simulink model "AFC_FFNN_trainbfg_60_60_60_Nor_July_15_Rep"  (R2021a)
settings: Solver=ode15s  StartTime=0.0  StopTime=T  MaxStep=.01  RelTol=1e-3
undefined symbols (not defined in the file): AF_sensor_tol, fault_time, fuel_inj_tol, kappa_tol, MAF_sensor_tol, pump_tol, tau_ww_tol, Ts, x_gain, x_offset, y_gain, y_offset
libraries: neural x185, dspsrcs4 x3
(part 2 of 8)

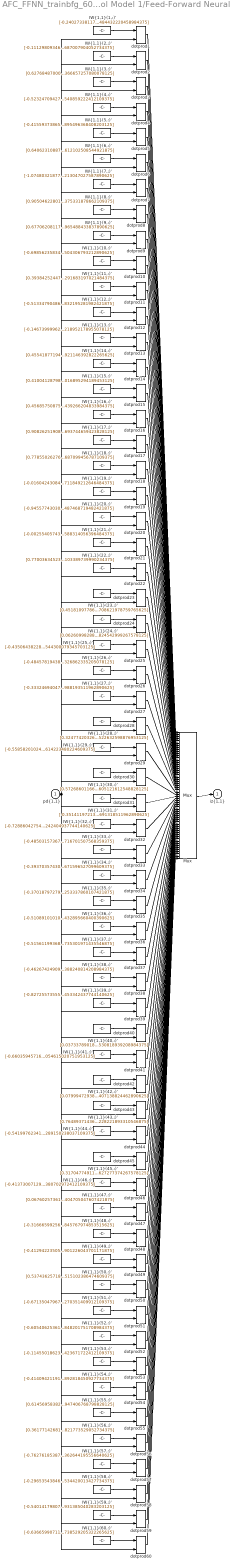
== system AFC_FFNN_trainbfg_60_60_60_Nor_July_15_Rep/Air Fuel Control Model 1/Feed-Forward Neural Network/Layer 1/IW{1,1} ==
  "pd{1,1}" : Inport  PortDimensions=4
      mask Display: e = 0.06;c1 = [120 230 180]/255;c2 = ([120 230 180]+0)/(256+128);c3 = ([120 230 180]+128)/(256+128);patch([0 1 1 0],[0 0 1 1],c1);patch([0 1 1 1-e 1-e 0+e],[0 0 1 1-e 0+e 0+e],c2);patch([0 0 1 1-e 0+e 0+e],[0 1 1 1-e 1-e 0+e],c3);plot([0 1 1 0 0],[0 0 1 1 0]);
  "IW{1,1}(1,:)'" : Constant  Value=[-0.2402733811760711102323284649173729121685028076171875;0.0584441094356973334100757710984908044338226318359375;-0.6963364088024845965918530055205337703227996826171875;-0.288781535204351680334866614430211484432220458984375]
      mask Display: e = 0.06;c1 = [120 150 230]/255;c2 = ([120 150 230]+0)/383;c3 = ([120 150 230]+128)/383;patch([0 1 1 0],[0 0 1 1],c1);patch([0 1 1 1-e 1-e 0+e],[0 0 1 1-e 0+e 0+e],c2);patch([0 0 1 1-e 0+e 0+e],[0 1 1 1-e 1-e 0+e],c3);plot([0 1 1 0 0],[0 0 1 1 0]);disp('Weights');
  "IW{1,1}(10,:)'" : Constant  Value=[-0.698562358345947043147816657437942922115325927734375;0.69054064531703496232495353979174979031085968017578125;-0.18905586459529022391734542907215654850006103515625;-0.91927275641961225804976720610284246504306793212890625]
      mask Display: e = 0.06;c1 = [120 150 230]/255;c2 = ([120 150 230]+0)/383;c3 = ([120 150 230]+128)/383;patch([0 1 1 0],[0 0 1 1],c1);patch([0 1 1 1-e 1-e 0+e],[0 0 1 1-e 0+e 0+e],c2);patch([0 0 1 1-e 0+e 0+e],[0 1 1 1-e 1-e 0+e],c3);plot([0 1 1 0 0],[0 0 1 1 0]);disp('Weights');
  "IW{1,1}(11,:)'" : Constant  Value=[0.39384252447863554724705181797617115080356597900390625;-0.0292738838791086024293530698514587129466235637664794921875;0.58197351258983232025201459691743366420269012451171875;0.8598468943954189480649574761628173291683197021484375]
      mask Display: e = 0.06;c1 = [120 150 230]/255;c2 = ([120 150 230]+0)/383;c3 = ([120 150 230]+128)/383;patch([0 1 1 0],[0 0 1 1],c1);patch([0 1 1 1-e 1-e 0+e],[0 0 1 1-e 0+e 0+e],c2);patch([0 0 1 1-e 0+e 0+e],[0 1 1 1-e 1-e 0+e],c3);plot([0 1 1 0 0],[0 0 1 1 0]);disp('Weights');
  "IW{1,1}(12,:)'" : Constant  Value=[-0.513347904862785586743711974122561514377593994140625;-0.869373002560909657887577850488014519214630126953125;0.72775650268875191617468090043985284864902496337890625;0.47288176623451583235890893774922005832195281982421875]
      mask Display: e = 0.06;c1 = [120 150 230]/255;c2 = ([120 150 230]+0)/383;c3 = ([120 150 230]+128)/383;patch([0 1 1 0],[0 0 1 1],c1);patch([0 1 1 1-e 1-e 0+e],[0 0 1 1-e 0+e 0+e],c2);patch([0 0 1 1-e 0+e 0+e],[0 1 1 1-e 1-e 0+e],c3);plot([0 1 1 0 0],[0 0 1 1 0]);disp('Weights');
  "IW{1,1}(13,:)'" : Constant  Value=[-0.1467399996214004131989128154600621201097965240478515625;-0.249808478302043723839886979476432316005229949951171875;0.507943904783524136092864864622242748737335205078125;0.71026397639314087228967764531262218952178955078125]
      mask Display: e = 0.06;c1 = [120 150 230]/255;c2 = ([120 150 230]+0)/383;c3 = ([120 150 230]+128)/383;patch([0 1 1 0],[0 0 1 1],c1);patch([0 1 1 1-e 1-e 0+e],[0 0 1 1-e 0+e 0+e],c2);patch([0 0 1 1-e 0+e 0+e],[0 1 1 1-e 1-e 0+e],c3);plot([0 1 1 0 0],[0 0 1 1 0]);disp('Weights');
  "IW{1,1}(14,:)'" : Constant  Value=[0.4554187719467928108230125872069038450717926025390625;0.411659817080715140225066761558991856873035430908203125;0.2102615703971319194298672528020688332617282867431640625;-0.322493540823335200773414044306264258921146392822265625]
      mask Display: e = 0.06;c1 = [120 150 230]/255;c2 = ([120 150 230]+0)/383;c3 = ([120 150 230]+128)/383;patch([0 1 1 0],[0 0 1 1],c1);patch([0 1 1 1-e 1-e 0+e],[0 0 1 1-e 0+e 0+e],c2);patch([0 0 1 1-e 0+e 0+e],[0 1 1 1-e 1-e 0+e],c3);plot([0 1 1 0 0],[0 0 1 1 0]);disp('Weights');
  "IW{1,1}(15,:)'" : Constant  Value=[0.410041287982604085726734410854987800121307373046875;0.531329072729679108277878185617737472057342529296875;0.441581495936325563178570519085042178630828857421875;0.7428199021330688101016903601703234016895294189453125]
      mask Display: e = 0.06;c1 = [120 150 230]/255;c2 = ([120 150 230]+0)/383;c3 = ([120 150 230]+128)/383;patch([0 1 1 0],[0 0 1 1],c1);patch([0 1 1 1-e 1-e 0+e],[0 0 1 1-e 0+e 0+e],c2);patch([0 0 1 1-e 0+e 0+e],[0 1 1 1-e 1-e 0+e],c3);plot([0 1 1 0 0],[0 0 1 1 0]);disp('Weights');
  "IW{1,1}(16,:)'" : Constant  Value=[0.45685750875504094192791626483085565268993377685546875;-0.465586840801124945965483448162558488547801971435546875;-0.9097857307732315490511609823442995548248291015625;0.056854430973618828859539320319527178071439266204833984375]
      mask Display: e = 0.06;c1 = [120 150 230]/255;c2 = ([120 150 230]+0)/383;c3 = ([120 150 230]+128)/383;patch([0 1 1 0],[0 0 1 1],c1);patch([0 1 1 1-e 1-e 0+e],[0 0 1 1-e 0+e 0+e],c2);patch([0 0 1 1-e 0+e 0+e],[0 1 1 1-e 1-e 0+e],c3);plot([0 1 1 0 0],[0 0 1 1 0]);disp('Weights');
  "IW{1,1}(17,:)'" : Constant  Value=[0.90826251908224531206315077724866569042205810546875;-0.168991405620153134492511526332236826419830322265625;-0.3326678975694663531470496309339068830013275146484375;-0.2185158166571838922465076393564231693744659423828125]
      mask Display: e = 0.06;c1 = [120 150 230]/255;c2 = ([120 150 230]+0)/383;c3 = ([120 150 230]+128)/383;patch([0 1 1 0],[0 0 1 1],c1);patch([0 1 1 1-e 1-e 0+e],[0 0 1 1-e 0+e 0+e],c2);patch([0 0 1 1-e 0+e 0+e],[0 1 1 1-e 1-e 0+e],c3);plot([0 1 1 0 0],[0 0 1 1 0]);disp('Weights');
  "IW{1,1}(18,:)'" : Constant  Value=[0.77855026276990724198867610539309680461883544921875;0.5494533878008895921851717503159306943416595458984375;-0.19968633757158349428806332070962525904178619384765625;0.057413702447717838983631821747621870599687099456787109375]
      mask Display: e = 0.06;c1 = [120 150 230]/255;c2 = ([120 150 230]+0)/383;c3 = ([120 150 230]+128)/383;patch([0 1 1 0],[0 0 1 1],c1);patch([0 1 1 1-e 1-e 0+e],[0 0 1 1-e 0+e 0+e],c2);patch([0 0 1 1-e 0+e 0+e],[0 1 1 1-e 1-e 0+e],c3);plot([0 1 1 0 0],[0 0 1 1 0]);disp('Weights');
  "IW{1,1}(19,:)'" : Constant  Value=[-0.01604243084496127791371833382072509266436100006103515625;0.7508500028717011165468875333317555487155914306640625;0.702339376844223206575179574429057538509368896484375;-0.96384498936832496696069938479922711849212646484375]
      mask Display: e = 0.06;c1 = [120 150 230]/255;c2 = ([120 150 230]+0)/383;c3 = ([120 150 230]+128)/383;patch([0 1 1 0],[0 0 1 1],c1);patch([0 1 1 1-e 1-e 0+e],[0 0 1 1-e 0+e 0+e],c2);patch([0 0 1 1-e 0+e 0+e],[0 1 1 1-e 1-e 0+e],c3);plot([0 1 1 0 0],[0 0 1 1 0]);disp('Weights');
  "IW{1,1}(2,:)'" : Constant  Value=[-0.11129809346802523040143029220416792668402194976806640625;1.19471297517650665298560852534137666225433349609375;0.8221228609018293997934279104811139404773712158203125;0.261811524571846143683018226511194370687007904052734375]
      mask Display: e = 0.06;c1 = [120 150 230]/255;c2 = ([120 150 230]+0)/383;c3 = ([120 150 230]+128)/383;patch([0 1 1 0],[0 0 1 1],c1);patch([0 1 1 1-e 1-e 0+e],[0 0 1 1-e 0+e 0+e],c2);patch([0 0 1 1-e 0+e 0+e],[0 1 1 1-e 1-e 0+e],c3);plot([0 1 1 0 0],[0 0 1 1 0]);disp('Weights');
  "IW{1,1}(20,:)'" : Constant  Value=[-0.945577430309771482797032149392180144786834716796875;-0.6815723884271618349117716206819750368595123291015625;0.3251297032677182841098328935913741588592529296875;-0.27675916067568884226801628756220452487468719482421875]
      mask Display: e = 0.06;c1 = [120 150 230]/255;c2 = ([120 150 230]+0)/383;c3 = ([120 150 230]+128)/383;patch([0 1 1 0],[0 0 1 1],c1);patch([0 1 1 1-e 1-e 0+e],[0 0 1 1-e 0+e 0+e],c2);patch([0 0 1 1-e 0+e 0+e],[0 1 1 1-e 1-e 0+e],c3);plot([0 1 1 0 0],[0 0 1 1 0]);disp('Weights');
  "IW{1,1}(21,:)'" : Constant  Value=[-0.0025540574341372016507756281811225562705658376216888427734375;-0.9119172902964922666768643466639332473278045654296875;-0.10602108765426902781126017316637444309890270233154296875;0.9466934496951624478100484338938258588314056396484375]
      mask Display: e = 0.06;c1 = [120 150 230]/255;c2 = ([120 150 230]+0)/383;c3 = ([120 150 230]+128)/383;patch([0 1 1 0],[0 0 1 1],c1);patch([0 1 1 1-e 1-e 0+e],[0 0 1 1-e 0+e 0+e],c2);patch([0 0 1 1-e 0+e 0+e],[0 1 1 1-e 1-e 0+e],c3);plot([0 1 1 0 0],[0 0 1 1 0]);disp('Weights');
  "IW{1,1}(22,:)'" : Constant  Value=[0.77003634523305664050241148288478143513202667236328125;0.5101538838642649675847451362642459571361541748046875;1.2853720282784777406703824453870765864849090576171875;-0.3114234464103569077764177563949488103389739990234375]
      mask Display: e = 0.06;c1 = [120 150 230]/255;c2 = ([120 150 230]+0)/383;c3 = ([120 150 230]+128)/383;patch([0 1 1 0],[0 0 1 1],c1);patch([0 1 1 1-e 1-e 0+e],[0 0 1 1-e 0+e 0+e],c2);patch([0 0 1 1-e 0+e 0+e],[0 1 1 1-e 1-e 0+e],c3);plot([0 1 1 0 0],[0 0 1 1 0]);disp('Weights');
  "IW{1,1}(23,:)'" : Constant  Value=[0.451810977860063023303638374272850342094898223876953125;0.97595879998877788086275586465490050613880157470703125;-1.0004027544089548751315987829002551734447479248046875;0.425110540617065046919975657147006131708621978759765625]
      mask Display: e = 0.06;c1 = [120 150 230]/255;c2 = ([120 150 230]+0)/383;c3 = ([120 150 230]+128)/383;patch([0 1 1 0],[0 0 1 1],c1);patch([0 1 1 1-e 1-e 0+e],[0 0 1 1-e 0+e 0+e],c2);patch([0 0 1 1-e 0+e 0+e],[0 1 1 1-e 1-e 0+e],c3);plot([0 1 1 0 0],[0 0 1 1 0]);disp('Weights');
  "IW{1,1}(24,:)'" : Constant  Value=[0.06260998288320009097507323758691200055181980133056640625;0.70118255617086788777925221438636071979999542236328125;-0.41558101347191478414089260695618577301502227783203125;-0.8023807819065560398286152121727354824542999267578125]
      mask Display: e = 0.06;c1 = [120 150 230]/255;c2 = ([120 150 230]+0)/383;c3 = ([120 150 230]+128)/383;patch([0 1 1 0],[0 0 1 1],c1);patch([0 1 1 1-e 1-e 0+e],[0 0 1 1-e 0+e 0+e],c2);patch([0 0 1 1-e 0+e 0+e],[0 1 1 1-e 1-e 0+e],c3);plot([0 1 1 0 0],[0 0 1 1 0]);disp('Weights');
  "IW{1,1}(25,:)'" : Constant  Value=[-0.43506438228140986712588755835895426571369171142578125;-1.10068797433876230940086315968073904514312744140625;0.58386265727177566464689562053536064922809600830078125;0.3360856882674394530141626091790385544300079345703125]
      mask Display: e = 0.06;c1 = [120 150 230]/255;c2 = ([120 150 230]+0)/383;c3 = ([120 150 230]+128)/383;patch([0 1 1 0],[0 0 1 1],c1);patch([0 1 1 1-e 1-e 0+e],[0 0 1 1-e 0+e 0+e],c2);patch([0 0 1 1-e 0+e 0+e],[0 1 1 1-e 1-e 0+e],c3);plot([0 1 1 0 0],[0 0 1 1 0]);disp('Weights');
  "IW{1,1}(26,:)'" : Constant  Value=[-0.484578194384843730091461111442185938358306884765625;0.08274506282760592246194875087894615717232227325439453125;0.266533819315904363378422203822992742061614990234375;-0.444300663044444654747877621048246510326862335205078125]
      mask Display: e = 0.06;c1 = [120 150 230]/255;c2 = ([120 150 230]+0)/383;c3 = ([120 150 230]+128)/383;patch([0 1 1 0],[0 0 1 1],c1);patch([0 1 1 1-e 1-e 0+e],[0 0 1 1-e 0+e 0+e],c2);patch([0 0 1 1-e 0+e 0+e],[0 1 1 1-e 1-e 0+e],c3);plot([0 1 1 0 0],[0 0 1 1 0]);disp('Weights');
  "IW{1,1}(27,:)'" : Constant  Value=[-0.333246940473589159381617719191126525402069091796875;0.620357973300408982453291173442266881465911865234375;-0.76705337279785357207373408527928404510021209716796875;0.93596136081508130022399427616619504988193511962890625]
      mask Display: e = 0.06;c1 = [120 150 230]/255;c2 = ([120 150 230]+0)/383;c3 = ([120 150 230]+128)/383;patch([0 1 1 0],[0 0 1 1],c1);patch([0 1 1 1-e 1-e 0+e],[0 0 1 1-e 0+e 0+e],c2);patch([0 0 1 1-e 0+e 0+e],[0 1 1 1-e 1-e 0+e],c3);plot([0 1 1 0 0],[0 0 1 1 0]);disp('Weights');
  "IW{1,1}(28,:)'" : Constant  Value=[0.324774203262355898313984425840317271649837493896484375;-0.321182382515287800917036520331748761236667633056640625;0.086974910188199194838176708799437619745731353759765625;0.51123135063906322006488380793598480522632598876953125]
      mask Display: e = 0.06;c1 = [120 150 230]/255;c2 = ([120 150 230]+0)/383;c3 = ([120 150 230]+128)/383;patch([0 1 1 0],[0 0 1 1],c1);patch([0 1 1 1-e 1-e 0+e],[0 0 1 1-e 0+e 0+e],c2);patch([0 0 1 1-e 0+e 0+e],[0 1 1 1-e 1-e 0+e],c3);plot([0 1 1 0 0],[0 0 1 1 0]);disp('Weights');
  "IW{1,1}(29,:)'" : Constant  Value=[-0.55858201024710985027610377073870040476322174072265625;0.75433144332418422539632274492760188877582550048828125;1.237291002285560548301646122126840054988861083984375;0.051530715501696099101192061198162264190614223480224609375]
      mask Display: e = 0.06;c1 = [120 150 230]/255;c2 = ([120 150 230]+0)/383;c3 = ([120 150 230]+128)/383;patch([0 1 1 0],[0 0 1 1],c1);patch([0 1 1 1-e 1-e 0+e],[0 0 1 1-e 0+e 0+e],c2);patch([0 0 1 1-e 0+e 0+e],[0 1 1 1-e 1-e 0+e],c3);plot([0 1 1 0 0],[0 0 1 1 0]);disp('Weights');
  "IW{1,1}(3,:)'" : Constant  Value=[0.62768487000840966771875173435546457767486572265625;-0.23395389022367485409859000355936586856842041015625;-0.7323866072763622891983459339826367795467376708984375;-0.43736410145401283244837031816132366657257080078125]
      mask Display: e = 0.06;c1 = [120 150 230]/255;c2 = ([120 150 230]+0)/383;c3 = ([120 150 230]+128)/383;patch([0 1 1 0],[0 0 1 1],c1);patch([0 1 1 1-e 1-e 0+e],[0 0 1 1-e 0+e 0+e],c2);patch([0 0 1 1-e 0+e 0+e],[0 1 1 1-e 1-e 0+e],c3);plot([0 1 1 0 0],[0 0 1 1 0]);disp('Weights');
  "IW{1,1}(30,:)'" : Constant  Value=[0.57268601166601029728298044574330560863018035888671875;0.5351151798944560056270347558893263339996337890625;0.6025777522967918908847195780253969132900238037109375;-0.4208352769974184059975641503115184605121612548828125]
      mask Display: e = 0.06;c1 = [120 150 230]/255;c2 = ([120 150 230]+0)/383;c3 = ([120 150 230]+128)/383;patch([0 1 1 0],[0 0 1 1],c1);patch([0 1 1 1-e 1-e 0+e],[0 0 1 1-e 0+e 0+e],c2);patch([0 0 1 1-e 0+e 0+e],[0 1 1 1-e 1-e 0+e],c3);plot([0 1 1 0 0],[0 0 1 1 0]);disp('Weights');
  "IW{1,1}(31,:)'" : Constant  Value=[-0.351411972139949624338584044380695559084415435791015625;-0.58862397289580592474322884299908764660358428955078125;0.405848519913738992048735099160694517195224761962890625;0.778774721855601370634758495725691318511962890625]
      mask Display: e = 0.06;c1 = [120 150 230]/255;c2 = ([120 150 230]+0)/383;c3 = ([120 150 230]+128)/383;patch([0 1 1 0],[0 0 1 1],c1);patch([0 1 1 1-e 1-e 0+e],[0 0 1 1-e 0+e 0+e],c2);patch([0 0 1 1-e 0+e 0+e],[0 1 1 1-e 1-e 0+e],c3);plot([0 1 1 0 0],[0 0 1 1 0]);disp('Weights');
  "IW{1,1}(32,:)'" : Constant  Value=[-0.7288604275436771917640044193831272423267364501953125;-0.996691557863663479821525470470078289508819580078125;0.433393450161783932994552515083341859281063079833984375;-0.99673661414379299827714930870570242404937744140625]
      mask Display: e = 0.06;c1 = [120 150 230]/255;c2 = ([120 150 230]+0)/383;c3 = ([120 150 230]+128)/383;patch([0 1 1 0],[0 0 1 1],c1);patch([0 1 1 1-e 1-e 0+e],[0 0 1 1-e 0+e 0+e],c2);patch([0 0 1 1-e 0+e 0+e],[0 1 1 1-e 1-e 0+e],c3);plot([0 1 1 0 0],[0 0 1 1 0]);disp('Weights');
  "IW{1,1}(33,:)'" : Constant  Value=[-0.485031573670599680525583607959561049938201904296875;0.611012222465525223213944627786986529827117919921875;-0.83546688891837372903381719879689626395702362060546875;-0.81775281563621859959312132559716701507568359375]
      mask Display: e = 0.06;c1 = [120 150 230]/255;c2 = ([120 150 230]+0)/383;c3 = ([120 150 230]+128)/383;patch([0 1 1 0],[0 0 1 1],c1);patch([0 1 1 1-e 1-e 0+e],[0 0 1 1-e 0+e 0+e],c2);patch([0 0 1 1-e 0+e 0+e],[0 1 1 1-e 1-e 0+e],c3);plot([0 1 1 0 0],[0 0 1 1 0]);disp('Weights');
  "IW{1,1}(34,:)'" : Constant  Value=[-0.3937035743010410815401201034546829760074615478515625;0.12437679182351264739470053655168158002197742462158203125;-0.1559704725434329919409037756850011646747589111328125;-0.377894968173168199765399322131997905671596527099609375]
      mask Display: e = 0.06;c1 = [120 150 230]/255;c2 = ([120 150 230]+0)/383;c3 = ([120 150 230]+128)/383;patch([0 1 1 0],[0 0 1 1],c1);patch([0 1 1 1-e 1-e 0+e],[0 0 1 1-e 0+e 0+e],c2);patch([0 0 1 1-e 0+e 0+e],[0 1 1 1-e 1-e 0+e],c3);plot([0 1 1 0 0],[0 0 1 1 0]);disp('Weights');
  "IW{1,1}(35,:)'" : Constant  Value=[-0.370187972793248276648370165275991894304752349853515625;-0.7998130855513536641154814788023941218852996826171875;0.359795410640817603376007127735647372901439666748046875;-0.7383023080329642606756124223466031253337860107421875]
      mask Display: e = 0.06;c1 = [120 150 230]/255;c2 = ([120 150 230]+0)/383;c3 = ([120 150 230]+128)/383;patch([0 1 1 0],[0 0 1 1],c1);patch([0 1 1 1-e 1-e 0+e],[0 0 1 1-e 0+e 0+e],c2);patch([0 0 1 1-e 0+e 0+e],[0 1 1 1-e 1-e 0+e],c3);plot([0 1 1 0 0],[0 0 1 1 0]);disp('Weights');
  "IW{1,1}(36,:)'" : Constant  Value=[-0.51089101010404203151438196073286235332489013671875;-0.56318994359729479537435281599755398929119110107421875;-0.377415197921292355776046179016702808439731597900390625;0.024662139600768552549769907500376575626432895660400390625]
      mask Display: e = 0.06;c1 = [120 150 230]/255;c2 = ([120 150 230]+0)/383;c3 = ([120 150 230]+128)/383;patch([0 1 1 0],[0 0 1 1],c1);patch([0 1 1 1-e 1-e 0+e],[0 0 1 1-e 0+e 0+e],c2);patch([0 0 1 1-e 0+e 0+e],[0 1 1 1-e 1-e 0+e],c3);plot([0 1 1 0 0],[0 0 1 1 0]);disp('Weights');
  "IW{1,1}(37,:)'" : Constant  Value=[-0.51561199368180066215927581652067601680755615234375;0.77000536182291334785787739747320301830768585205078125;0.29882660214653433694564910183544270694255828857421875;0.04938437783104136780121251604214194230735301971435546875]
      mask Display: e = 0.06;c1 = [120 150 230]/255;c2 = ([120 150 230]+0)/383;c3 = ([120 150 230]+128)/383;patch([0 1 1 0],[0 0 1 1],c1);patch([0 1 1 1-e 1-e 0+e],[0 0 1 1-e 0+e 0+e],c2);patch([0 0 1 1-e 0+e 0+e],[0 1 1 1-e 1-e 0+e],c3);plot([0 1 1 0 0],[0 0 1 1 0]);disp('Weights');
  "IW{1,1}(38,:)'" : Constant  Value=[-0.462674249097232370697696524075581692159175872802734375;-0.20404535875965346125582300373935140669345855712890625;-0.643589688538109161441980177187360823154449462890625;0.172530502878537050914786732391803525388240814208984375]
      mask Display: e = 0.06;c1 = [120 150 230]/255;c2 = ([120 150 230]+0)/383;c3 = ([120 150 230]+128)/383;patch([0 1 1 0],[0 0 1 1],c1);patch([0 1 1 1-e 1-e 0+e],[0 0 1 1-e 0+e 0+e],c2);patch([0 0 1 1-e 0+e 0+e],[0 1 1 1-e 1-e 0+e],c3);plot([0 1 1 0 0],[0 0 1 1 0]);disp('Weights');
  "IW{1,1}(39,:)'" : Constant  Value=[-0.827255735558199756241037903237156569957733154296875;0.31768520899595087403355364585877396166324615478515625;-0.26820571117561098350989823302370496094226837158203125;0.78370361390073883800511111985542811453342437744140625]
      mask Display: e = 0.06;c1 = [120 150 230]/255;c2 = ([120 150 230]+0)/383;c3 = ([120 150 230]+128)/383;patch([0 1 1 0],[0 0 1 1],c1);patch([0 1 1 1-e 1-e 0+e],[0 0 1 1-e 0+e 0+e],c2);patch([0 0 1 1-e 0+e 0+e],[0 1 1 1-e 1-e 0+e],c3);plot([0 1 1 0 0],[0 0 1 1 0]);disp('Weights');
  "IW{1,1}(4,:)'" : Constant  Value=[-0.5232470942791049850484341732226312160491943359375;-0.6811423805727827573974764163722284138202667236328125;-0.610543497321023753698909786180593073368072509765625;-0.224003810896950650288772521889768540859222412109375]
      mask Display: e = 0.06;c1 = [120 150 230]/255;c2 = ([120 150 230]+0)/383;c3 = ([120 150 230]+128)/383;patch([0 1 1 0],[0 0 1 1],c1);patch([0 1 1 1-e 1-e 0+e],[0 0 1 1-e 0+e 0+e],c2);patch([0 0 1 1-e 0+e 0+e],[0 1 1 1-e 1-e 0+e],c3);plot([0 1 1 0 0],[0 0 1 1 0]);disp('Weights');
  "IW{1,1}(40,:)'" : Constant  Value=[0.0373378901805889729104137586546130478382110595703125;0.8513626591803109544542849107529036700725555419921875;-0.9283781102192214529367220166022889316082000732421875;-0.250683731280675115016265408485196530818939208984375]
      mask Display: e = 0.06;c1 = [120 150 230]/255;c2 = ([120 150 230]+0)/383;c3 = ([120 150 230]+128)/383;patch([0 1 1 0],[0 0 1 1],c1);patch([0 1 1 1-e 1-e 0+e],[0 0 1 1-e 0+e 0+e],c2);patch([0 0 1 1-e 0+e 0+e],[0 1 1 1-e 1-e 0+e],c3);plot([0 1 1 0 0],[0 0 1 1 0]);disp('Weights');
  "IW{1,1}(41,:)'" : Constant  Value=[-0.660359457166579399967076824395917356014251708984375;-0.9795941991072105725635310591314919292926788330078125;-0.922451670193998207736285621649585664272308349609375;-0.87504814362874316913121219840832054615020751953125]
      mask Display: e = 0.06;c1 = [120 150 230]/255;c2 = ([120 150 230]+0)/383;c3 = ([120 150 230]+128)/383;patch([0 1 1 0],[0 0 1 1],c1);patch([0 1 1 1-e 1-e 0+e],[0 0 1 1-e 0+e 0+e],c2);patch([0 0 1 1-e 0+e 0+e],[0 1 1 1-e 1-e 0+e],c3);plot([0 1 1 0 0],[0 0 1 1 0]);disp('Weights');
  "IW{1,1}(42,:)'" : Constant  Value=[0.0799947293830058914210212606121785938739776611328125;-0.01554714821110536604464869014918804168701171875;0.9410230983615124333852008930989541113376617431640625;-0.4172880678448687152837237590574659407138824462890625]
      mask Display: e = 0.06;c1 = [120 150 230]/255;c2 = ([120 150 230]+0)/383;c3 = ([120 150 230]+128)/383;patch([0 1 1 0],[0 0 1 1],c1);patch([0 1 1 1-e 1-e 0+e],[0 0 1 1-e 0+e 0+e],c2);patch([0 0 1 1-e 0+e 0+e],[0 1 1 1-e 1-e 0+e],c3);plot([0 1 1 0 0],[0 0 1 1 0]);disp('Weights');
  "IW{1,1}(43,:)'" : Constant  Value=[0.7648937143639376046166944433934986591339111328125;-0.79666736296628493096960710317944176495075225830078125;0.2269171319430184630139279988725320436060428619384765625;0.312073469378814916108666466243448667228221893310546875]
      mask Display: e = 0.06;c1 = [120 150 230]/255;c2 = ([120 150 230]+0)/383;c3 = ([120 150 230]+128)/383;patch([0 1 1 0],[0 0 1 1],c1);patch([0 1 1 1-e 1-e 0+e],[0 0 1 1-e 0+e 0+e],c2);patch([0 0 1 1-e 0+e 0+e],[0 1 1 1-e 1-e 0+e],c3);plot([0 1 1 0 0],[0 0 1 1 0]);disp('Weights');
  "IW{1,1}(44,:)'" : Constant  Value=[-0.54199762341520685282603153609670698642730712890625;-0.6779396341603811659837219849578104913234710693359375;-0.0205716676017042576773974360548891127109527587890625;-0.2567857149437704489258749163127504289150238037109375]
      mask Display: e = 0.06;c1 = [120 150 230]/255;c2 = ([120 150 230]+0)/383;c3 = ([120 150 230]+128)/383;patch([0 1 1 0],[0 0 1 1],c1);patch([0 1 1 1-e 1-e 0+e],[0 0 1 1-e 0+e 0+e],c2);patch([0 0 1 1-e 0+e 0+e],[0 1 1 1-e 1-e 0+e],c3);plot([0 1 1 0 0],[0 0 1 1 0]);disp('Weights');
  "IW{1,1}(45,:)'" : Constant  Value=[0.317047749110300036701204362543649040162563323974609375;-0.49922870142301134510631754892528988420963287353515625;0.6173835365827649024339507377590052783489227294921875;-0.86470722989512360801001022991840727627277374267578125]
      mask Display: e = 0.06;c1 = [120 150 230]/255;c2 = ([120 150 230]+0)/383;c3 = ([120 150 230]+128)/383;patch([0 1 1 0],[0 0 1 1],c1);patch([0 1 1 1-e 1-e 0+e],[0 0 1 1-e 0+e 0+e],c2);patch([0 0 1 1-e 0+e 0+e],[0 1 1 1-e 1-e 0+e],c3);plot([0 1 1 0 0],[0 0 1 1 0]);disp('Weights');
  "IW{1,1}(46,:)'" : Constant  Value=[-0.41373007129052374875044506552512757480144500732421875;-0.4215260072473479002752583255642093718051910400390625;1.0491347537545305801387485189479775726795196533203125;-0.5364939166190045849447187720215879380702972412109375]
      mask Display: e = 0.06;c1 = [120 150 230]/255;c2 = ([120 150 230]+0)/383;c3 = ([120 150 230]+128)/383;patch([0 1 1 0],[0 0 1 1],c1);patch([0 1 1 1-e 1-e 0+e],[0 0 1 1-e 0+e 0+e],c2);patch([0 0 1 1-e 0+e 0+e],[0 1 1 1-e 1-e 0+e],c3);plot([0 1 1 0 0],[0 0 1 1 0]);disp('Weights');
  "IW{1,1}(47,:)'" : Constant  Value=[0.06760257361956799326829781193737289868295192718505859375;0.94355551412375093800477543481974862515926361083984375;-0.1792802164963338551473270854330621659755706787109375;-0.50551442944941982204909436404705047607421875]
      mask Display: e = 0.06;c1 = [120 150 230]/255;c2 = ([120 150 230]+0)/383;c3 = ([120 150 230]+128)/383;patch([0 1 1 0],[0 0 1 1],c1);patch([0 1 1 1-e 1-e 0+e],[0 0 1 1-e 0+e 0+e],c2);patch([0 0 1 1-e 0+e 0+e],[0 1 1 1-e 1-e 0+e],c3);plot([0 1 1 0 0],[0 0 1 1 0]);disp('Weights');
  "IW{1,1}(48,:)'" : Constant  Value=[-0.31666599256054206446009402498020790517330169677734375;-0.54546754033202649036837783569353632628917694091796875;0.66177681360233808760540341609157621860504150390625;-0.1927224913495736713375805493342340923845767974853515625]
      mask Display: e = 0.06;c1 = [120 150 230]/255;c2 = ([120 150 230]+0)/383;c3 = ([120 150 230]+128)/383;patch([0 1 1 0],[0 0 1 1],c1);patch([0 1 1 1-e 1-e 0+e],[0 0 1 1-e 0+e 0+e],c2);patch([0 0 1 1-e 0+e 0+e],[0 1 1 1-e 1-e 0+e],c3);plot([0 1 1 0 0],[0 0 1 1 0]);disp('Weights');
  "IW{1,1}(49,:)'" : Constant  Value=[-0.4129422350583700218606963971978984773159027099609375;-0.53958913236859107342979768873192369937896728515625;-0.9294797333998643384944671197445131838321685791015625;-0.886228284649959174856803656439296901226043701171875]
      mask Display: e = 0.06;c1 = [120 150 230]/255;c2 = ([120 150 230]+0)/383;c3 = ([120 150 230]+128)/383;patch([0 1 1 0],[0 0 1 1],c1);patch([0 1 1 1-e 1-e 0+e],[0 0 1 1-e 0+e 0+e],c2);patch([0 0 1 1-e 0+e 0+e],[0 1 1 1-e 1-e 0+e],c3);plot([0 1 1 0 0],[0 0 1 1 0]);disp('Weights');
  "IW{1,1}(5,:)'" : Constant  Value=[-0.415593738655633260226096581391175277531147003173828125;0.276190321120120152453836226413841359317302703857421875;0.362457390752062291738866406376473605632781982421875;0.53759792107391046744879758989554829895496368408203125]
      mask Display: e = 0.06;c1 = [120 150 230]/255;c2 = ([120 150 230]+0)/383;c3 = ([120 150 230]+128)/383;patch([0 1 1 0],[0 0 1 1],c1);patch([0 1 1 1-e 1-e 0+e],[0 0 1 1-e 0+e 0+e],c2);patch([0 0 1 1-e 0+e 0+e],[0 1 1 1-e 1-e 0+e],c3);plot([0 1 1 0 0],[0 0 1 1 0]);disp('Weights');
  "IW{1,1}(50,:)'" : Constant  Value=[0.53743625718462728624302826574421487748622894287109375;0.75654339789962576912074609936098568141460418701171875;-0.76269183869095502625867766255396418273448944091796875;0.87024611396621798231620914521045051515102386474609375]
      mask Display: e = 0.06;c1 = [120 150 230]/255;c2 = ([120 150 230]+0)/383;c3 = ([120 150 230]+128)/383;patch([0 1 1 0],[0 0 1 1],c1);patch([0 1 1 1-e 1-e 0+e],[0 0 1 1-e 0+e 0+e],c2);patch([0 0 1 1-e 0+e 0+e],[0 1 1 1-e 1-e 0+e],c3);plot([0 1 1 0 0],[0 0 1 1 0]);disp('Weights');
  "IW{1,1}(51,:)'" : Constant  Value=[-0.67135047967206429309072746036690659821033477783203125;0.007742226950816807722055568063979080761782824993133544921875;0.7478663580711411018597800648421980440616607666015625;-0.25103774691161750975965105681098066270351409912109375]
      mask Display: e = 0.06;c1 = [120 150 230]/255;c2 = ([120 150 230]+0)/383;c3 = ([120 150 230]+128)/383;patch([0 1 1 0],[0 0 1 1],c1);patch([0 1 1 1-e 1-e 0+e],[0 0 1 1-e 0+e 0+e],c2);patch([0 0 1 1-e 0+e 0+e],[0 1 1 1-e 1-e 0+e],c3);plot([0 1 1 0 0],[0 0 1 1 0]);disp('Weights');
  "IW{1,1}(52,:)'" : Constant  Value=[-0.60540625361792554937068189246929250657558441162109375;-0.22089027460524679469244802021421492099761962890625;0.926954408382917538489209619001485407352447509765625;-0.60630353264879432995115848825662396848201751708984375]
      mask Display: e = 0.06;c1 = [120 150 230]/255;c2 = ([120 150 230]+0)/383;c3 = ([120 150 230]+128)/383;patch([0 1 1 0],[0 0 1 1],c1);patch([0 1 1 1-e 1-e 0+e],[0 0 1 1-e 0+e 0+e],c2);patch([0 0 1 1-e 0+e 0+e],[0 1 1 1-e 1-e 0+e],c3);plot([0 1 1 0 0],[0 0 1 1 0]);disp('Weights');
  "IW{1,1}(53,:)'" : Constant  Value=[-0.1145501862381349267305807870798162184655666351318359375;0.32495452919710221539872918583569116890430450439453125;-0.6290532885715425237549425219185650348663330078125;-0.5938641277619804981213746941648423671722412109375]
      mask Display: e = 0.06;c1 = [120 150 230]/255;c2 = ([120 150 230]+0)/383;c3 = ([120 150 230]+128)/383;patch([0 1 1 0],[0 0 1 1],c1);patch([0 1 1 1-e 1-e 0+e],[0 0 1 1-e 0+e 0+e],c2);patch([0 0 1 1-e 0+e 0+e],[0 1 1 1-e 1-e 0+e],c3);plot([0 1 1 0 0],[0 0 1 1 0]);disp('Weights');
  "IW{1,1}(54,:)'" : Constant  Value=[-0.41409421191680595430995026617893017828464508056640625;-0.2467866136246865405023953599084052257239818572998046875;-0.79462668143061987446884586461237631738185882568359375;-0.313287341288275678063968143760575912892818450927734375]
      mask Display: e = 0.06;c1 = [120 150 230]/255;c2 = ([120 150 230]+0)/383;c3 = ([120 150 230]+128)/383;patch([0 1 1 0],[0 0 1 1],c1);patch([0 1 1 1-e 1-e 0+e],[0 0 1 1-e 0+e 0+e],c2);patch([0 0 1 1-e 0+e 0+e],[0 1 1 1-e 1-e 0+e],c3);plot([0 1 1 0 0],[0 0 1 1 0]);disp('Weights');
  "IW{1,1}(55,:)'" : Constant  Value=[0.61456958382935999996021791957900859415531158447265625;0.77906840401004207041779636710998602211475372314453125;-0.05469814453797294806491890994948334991931915283203125;-0.75170105282260479828693178205867297947406768798828125]
      mask Display: e = 0.06;c1 = [120 150 230]/255;c2 = ([120 150 230]+0)/383;c3 = ([120 150 230]+128)/383;patch([0 1 1 0],[0 0 1 1],c1);patch([0 1 1 1-e 1-e 0+e],[0 0 1 1-e 0+e 0+e],c2);patch([0 0 1 1-e 0+e 0+e],[0 1 1 1-e 1-e 0+e],c3);plot([0 1 1 0 0],[0 0 1 1 0]);disp('Weights');
  "IW{1,1}(56,:)'" : Constant  Value=[0.36177142681524776524071285166428424417972564697265625;0.96972691231273155931802421036991290748119354248046875;0.60073223464636893442758491801214404404163360595703125;-0.2408131518882239419099278165958821773529052734375]
      mask Display: e = 0.06;c1 = [120 150 230]/255;c2 = ([120 150 230]+0)/383;c3 = ([120 150 230]+128)/383;patch([0 1 1 0],[0 0 1 1],c1);patch([0 1 1 1-e 1-e 0+e],[0 0 1 1-e 0+e 0+e],c2);patch([0 0 1 1-e 0+e 0+e],[0 1 1 1-e 1-e 0+e],c3);plot([0 1 1 0 0],[0 0 1 1 0]);disp('Weights');
  "IW{1,1}(57,:)'" : Constant  Value=[-0.76276185387199835208349441018071956932544708251953125;-0.2421375945745911362205760042343172244727611541748046875;-0.401158995256248374072782780785928480327129364013671875;-0.949215891246782295098682880052365362644195556640625]
      mask Display: e = 0.06;c1 = [120 150 230]/255;c2 = ([120 150 230]+0)/383;c3 = ([120 150 230]+128)/383;patch([0 1 1 0],[0 0 1 1],c1);patch([0 1 1 1-e 1-e 0+e],[0 0 1 1-e 0+e 0+e],c2);patch([0 0 1 1-e 0+e 0+e],[0 1 1 1-e 1-e 0+e],c3);plot([0 1 1 0 0],[0 0 1 1 0]);disp('Weights');
  "IW{1,1}(58,:)'" : Constant  Value=[-0.2965354384694702805091992559027858078479766845703125;-0.61045069302128229793424907256849110126495361328125;-0.5856975978713683250731492080376483500003814697265625;-0.6917989449578152427733357399119995534420013427734375]
      mask Display: e = 0.06;c1 = [120 150 230]/255;c2 = ([120 150 230]+0)/383;c3 = ([120 150 230]+128)/383;patch([0 1 1 0],[0 0 1 1],c1);patch([0 1 1 1-e 1-e 0+e],[0 0 1 1-e 0+e 0+e],c2);patch([0 0 1 1-e 0+e 0+e],[0 1 1 1-e 1-e 0+e],c3);plot([0 1 1 0 0],[0 0 1 1 0]);disp('Weights');
  "IW{1,1}(59,:)'" : Constant  Value=[-0.5401417980790166328830537167959846556186676025390625;0.9439268925093784456947787475655786693096160888671875;-0.734518353919943134400227791047655045986175537109375;0.1330476894397207843212527222931385040283203125]
      mask Display: e = 0.06;c1 = [120 150 230]/255;c2 = ([120 150 230]+0)/383;c3 = ([120 150 230]+128)/383;patch([0 1 1 0],[0 0 1 1],c1);patch([0 1 1 1-e 1-e 0+e],[0 0 1 1-e 0+e 0+e],c2);patch([0 0 1 1-e 0+e 0+e],[0 1 1 1-e 1-e 0+e],c3);plot([0 1 1 0 0],[0 0 1 1 0]);disp('Weights');
  "IW{1,1}(6,:)'" : Constant  Value=[0.640623108875285840468905007583089172840118408203125;0.25429238087652727973164701325003989040851593017578125;-0.6911364053373347804409831951488740742206573486328125;0.90534245876376484574166170204989612102508544921875]
      mask Display: e = 0.06;c1 = [120 150 230]/255;c2 = ([120 150 230]+0)/383;c3 = ([120 150 230]+128)/383;patch([0 1 1 0],[0 0 1 1],c1);patch([0 1 1 1-e 1-e 0+e],[0 0 1 1-e 0+e 0+e],c2);patch([0 0 1 1-e 0+e 0+e],[0 1 1 1-e 1-e 0+e],c3);plot([0 1 1 0 0],[0 0 1 1 0]);disp('Weights');
  "IW{1,1}(60,:)'" : Constant  Value=[-0.63665990711108555455410851209308020770549774169921875;0.3853724837622551913085544583736918866634368896484375;0.09015503608517803912913990416200249455869197845458984375;0.29674320000994447443787294105277396738529205322265625]
      mask Display: e = 0.06;c1 = [120 150 230]/255;c2 = ([120 150 230]+0)/383;c3 = ([120 150 230]+128)/383;patch([0 1 1 0],[0 0 1 1],c1);patch([0 1 1 1-e 1-e 0+e],[0 0 1 1-e 0+e 0+e],c2);patch([0 0 1 1-e 0+e 0+e],[0 1 1 1-e 1-e 0+e],c3);plot([0 1 1 0 0],[0 0 1 1 0]);disp('Weights');
  "IW{1,1}(7,:)'" : Constant  Value=[-1.074803218774835311677406934904865920543670654296875;0.01867309465761823883411807400989346206188201904296875;0.544587811760389950421767935040406882762908935546875;-0.70469709872743957479457321824156679213047027587890625]
      mask Display: e = 0.06;c1 = [120 150 230]/255;c2 = ([120 150 230]+0)/383;c3 = ([120 150 230]+128)/383;patch([0 1 1 0],[0 0 1 1],c1);patch([0 1 1 1-e 1-e 0+e],[0 0 1 1-e 0+e 0+e],c2);patch([0 0 1 1-e 0+e 0+e],[0 1 1 1-e 1-e 0+e],c3);plot([0 1 1 0 0],[0 0 1 1 0]);disp('Weights');
  "IW{1,1}(8,:)'" : Constant  Value=[0.9050462280178359630866680163308046758174896240234375;-0.464526846162018614005972949598799459636211395263671875;-0.633686546389868876616446868865750730037689208984375;-0.484820283957884290426676443530595861375331878662109375]
      mask Display: e = 0.06;c1 = [120 150 230]/255;c2 = ([120 150 230]+0)/383;c3 = ([120 150 230]+128)/383;patch([0 1 1 0],[0 0 1 1],c1);patch([0 1 1 1-e 1-e 0+e],[0 0 1 1-e 0+e 0+e],c2);patch([0 0 1 1-e 0+e 0+e],[0 1 1 1-e 1-e 0+e],c3);plot([0 1 1 0 0],[0 0 1 1 0]);disp('Weights');
  "IW{1,1}(9,:)'" : Constant  Value=[0.67706208117781663258227808910305611789226531982421875;0.2374544377168311959369617625270620919764041900634765625;0.1842653102627499206445094159789732657372951507568359375;-0.366059443203293088942018584930337965488433837890625]
      mask Display: e = 0.06;c1 = [120 150 230]/255;c2 = ([120 150 230]+0)/383;c3 = ([120 150 230]+128)/383;patch([0 1 1 0],[0 0 1 1],c1);patch([0 1 1 1-e 1-e 0+e],[0 0 1 1-e 0+e 0+e],c2);patch([0 0 1 1-e 0+e 0+e],[0 1 1 1-e 1-e 0+e],c3);plot([0 1 1 0 0],[0 0 1 1 0]);disp('Weights');
  Mux : Mux  Inputs=60
      mask Display: e = 0.06;c1 = [120 150 230]/255;c2 = ([120 150 230]+0)/383;c3 = ([120 150 230]+128)/383;patch([0 1 1 0],[0 0 1 1],c1);patch([0 1 1 1-e 1-e 0+e],[0 0 1 1-e 0+e 0+e],c2);patch([0 0 1 1-e 0+e 0+e],[0 1 1 1-e 1-e 0+e],c3);plot([0 1 1 0 0],[0 0 1 1 0]);disp('Mux');
  dotprod{1..60} (60 alike) : neural/Weight Functions/dotprod
  "iz{1,1}" : Outport
      mask Display: e = 0.06;c1 = [120 230 180]/255;c2 = ([120 230 180]+0)/(256+128);c3 = ([120 230 180]+128)/(256+128);patch([0 1 1 0],[0 0 1 1],c1);patch([0 1 1 1-e 1-e 0+e],[0 0 1 1-e 0+e 0+e],c2);patch([0 0 1 1-e 0+e 0+e],[0 1 1 1-e 1-e 0+e],c3);plot([0 1 1 0 0],[0 0 1 1 0]);
  wires:
  Mux/1 -> "iz{1,1}"/1
  dotprod60/1 -> Mux/60
  "IW{1,1}(60,:)'"/1 -> dotprod60/1
  dotprod59/1 -> Mux/59
  "IW{1,1}(59,:)'"/1 -> dotprod59/1
  dotprod58/1 -> Mux/58
  "IW{1,1}(58,:)'"/1 -> dotprod58/1
  dotprod57/1 -> Mux/57
  "IW{1,1}(57,:)'"/1 -> dotprod57/1
  dotprod56/1 -> Mux/56
  "IW{1,1}(56,:)'"/1 -> dotprod56/1
  dotprod55/1 -> Mux/55
  "IW{1,1}(55,:)'"/1 -> dotprod55/1
  dotprod54/1 -> Mux/54
  "IW{1,1}(54,:)'"/1 -> dotprod54/1
  dotprod53/1 -> Mux/53
  "IW{1,1}(53,:)'"/1 -> dotprod53/1
  dotprod52/1 -> Mux/52
  "IW{1,1}(52,:)'"/1 -> dotprod52/1
  dotprod51/1 -> Mux/51
  "IW{1,1}(51,:)'"/1 -> dotprod51/1
  dotprod50/1 -> Mux/50
  "IW{1,1}(50,:)'"/1 -> dotprod50/1
  dotprod49/1 -> Mux/49
  "IW{1,1}(49,:)'"/1 -> dotprod49/1
  dotprod48/1 -> Mux/48
  "IW{1,1}(48,:)'"/1 -> dotprod48/1
  dotprod47/1 -> Mux/47
  "IW{1,1}(47,:)'"/1 -> dotprod47/1
  dotprod46/1 -> Mux/46
  "IW{1,1}(46,:)'"/1 -> dotprod46/1
  dotprod45/1 -> Mux/45
  "IW{1,1}(45,:)'"/1 -> dotprod45/1
  dotprod44/1 -> Mux/44
  "IW{1,1}(44,:)'"/1 -> dotprod44/1
  dotprod43/1 -> Mux/43
  "IW{1,1}(43,:)'"/1 -> dotprod43/1
  dotprod42/1 -> Mux/42
  "IW{1,1}(42,:)'"/1 -> dotprod42/1
  dotprod41/1 -> Mux/41
  "IW{1,1}(41,:)'"/1 -> dotprod41/1
  dotprod40/1 -> Mux/40
  "IW{1,1}(40,:)'"/1 -> dotprod40/1
  dotprod39/1 -> Mux/39
  "IW{1,1}(39,:)'"/1 -> dotprod39/1
  dotprod38/1 -> Mux/38
  "IW{1,1}(38,:)'"/1 -> dotprod38/1
  dotprod37/1 -> Mux/37
  "IW{1,1}(37,:)'"/1 -> dotprod37/1
  dotprod36/1 -> Mux/36
  "IW{1,1}(36,:)'"/1 -> dotprod36/1
  dotprod35/1 -> Mux/35
  "IW{1,1}(35,:)'"/1 -> dotprod35/1
  dotprod34/1 -> Mux/34
  "IW{1,1}(34,:)'"/1 -> dotprod34/1
  dotprod33/1 -> Mux/33
  "IW{1,1}(33,:)'"/1 -> dotprod33/1
  dotprod32/1 -> Mux/32
  "IW{1,1}(32,:)'"/1 -> dotprod32/1
  dotprod31/1 -> Mux/31
  "IW{1,1}(31,:)'"/1 -> dotprod31/1
  dotprod30/1 -> Mux/30
  "IW{1,1}(30,:)'"/1 -> dotprod30/1
  dotprod29/1 -> Mux/29
  "IW{1,1}(29,:)'"/1 -> dotprod29/1
  dotprod28/1 -> Mux/28
  "IW{1,1}(28,:)'"/1 -> dotprod28/1
  dotprod27/1 -> Mux/27
  "IW{1,1}(27,:)'"/1 -> dotprod27/1
  dotprod26/1 -> Mux/26
  "IW{1,1}(26,:)'"/1 -> dotprod26/1
  dotprod25/1 -> Mux/25
  "IW{1,1}(25,:)'"/1 -> dotprod25/1
  dotprod24/1 -> Mux/24
  "IW{1,1}(24,:)'"/1 -> dotprod24/1
  dotprod23/1 -> Mux/23
  "IW{1,1}(23,:)'"/1 -> dotprod23/1
  dotprod22/1 -> Mux/22
  "IW{1,1}(22,:)'"/1 -> dotprod22/1
  dotprod21/1 -> Mux/21
  "IW{1,1}(21,:)'"/1 -> dotprod21/1
  dotprod20/1 -> Mux/20
  "IW{1,1}(20,:)'"/1 -> dotprod20/1
  dotprod19/1 -> Mux/19
  "IW{1,1}(19,:)'"/1 -> dotprod19/1
  dotprod18/1 -> Mux/18
  "IW{1,1}(18,:)'"/1 -> dotprod18/1
  dotprod17/1 -> Mux/17
  "IW{1,1}(17,:)'"/1 -> dotprod17/1
  dotprod16/1 -> Mux/16
  "IW{1,1}(16,:)'"/1 -> dotprod16/1
  dotprod15/1 -> Mux/15
  "IW{1,1}(15,:)'"/1 -> dotprod15/1
  dotprod14/1 -> Mux/14
  "IW{1,1}(14,:)'"/1 -> dotprod14/1
  dotprod13/1 -> Mux/13
  "IW{1,1}(13,:)'"/1 -> dotprod13/1
  dotprod12/1 -> Mux/12
  "IW{1,1}(12,:)'"/1 -> dotprod12/1
  dotprod11/1 -> Mux/11
  "IW{1,1}(11,:)'"/1 -> dotprod11/1
  dotprod10/1 -> Mux/10
  "IW{1,1}(10,:)'"/1 -> dotprod10/1
  dotprod9/1 -> Mux/9
  "IW{1,1}(9,:)'"/1 -> dotprod9/1
  dotprod8/1 -> Mux/8
  "IW{1,1}(8,:)'"/1 -> dotprod8/1
  dotprod7/1 -> Mux/7
  "IW{1,1}(7,:)'"/1 -> dotprod7/1
  dotprod6/1 -> Mux/6
  "IW{1,1}(6,:)'"/1 -> dotprod6/1
  dotprod5/1 -> Mux/5
  "IW{1,1}(5,:)'"/1 -> dotprod5/1
  dotprod4/1 -> Mux/4
  "IW{1,1}(4,:)'"/1 -> dotprod4/1
  dotprod3/1 -> Mux/3
  "IW{1,1}(3,:)'"/1 -> dotprod3/1
  dotprod2/1 -> Mux/2
  "IW{1,1}(2,:)'"/1 -> dotprod2/1
  dotprod1/1 -> Mux/1
  "pd{1,1}"/1 -> dotprod60/2, dotprod59/2, dotprod58/2, dotprod57/2, dotprod56/2, dotprod55/2, dotprod54/2, dotprod53/2, dotprod52/2, dotprod51/2, dotprod50/2, dotprod49/2, dotprod48/2, dotprod47/2, dotprod46/2, dotprod45/2, dotprod44/2, dotprod43/2, dotprod42/2, dotprod41/2, dotprod40/2, dotprod39/2, dotprod38/2, dotprod37/2, dotprod36/2, dotprod35/2, dotprod34/2, dotprod33/2, dotprod32/2, dotprod31/2, dotprod30/2, dotprod29/2, dotprod28/2, dotprod27/2, dotprod26/2, dotprod25/2, dotprod24/2, dotprod23/2, dotprod22/2, dotprod21/2, dotprod20/2, dotprod19/2, dotprod18/2, dotprod17/2, dotprod16/2, dotprod15/2, dotprod14/2, dotprod13/2, dotprod12/2, dotprod11/2, dotprod10/2, dotprod9/2, dotprod8/2, dotprod7/2, dotprod6/2, dotprod5/2, dotprod4/2, dotprod3/2, dotprod2/2, dotprod1/2
  "IW{1,1}(1,:)'"/1 -> dotprod1/1

== system AFC_FFNN_trainbfg_60_60_60_Nor_July_15_Rep/Air Fuel Control Model 1/Feed-Forward Neural Network/Layer 2/Delays 1 ==
  "p{2}" : Inport  PortDimensions=60
      mask Display: e = 0.06;c1 = [120 230 180]/255;c2 = ([120 230 180]+0)/(256+128);c3 = ([120 230 180]+128)/(256+128);patch([0 1 1 0],[0 0 1 1],c1);patch([0 1 1 1-e 1-e 0+e],[0 0 1 1-e 0+e 0+e],c2);patch([0 0 1 1-e 0+e 0+e],[0 1 1 1-e 1-e 0+e],c3);plot([0 1 1 0 0],[0 0 1 1 0]);
  mux : Mux  Inputs=1
      mask Display: e = 0.06;c1 = [120 150 230]/255;c2 = ([120 150 230]+0)/383;c3 = ([120 150 230]+128)/383;patch([0 1 1 0],[0 0 1 1],c1);patch([0 1 1 1-e 1-e 0+e],[0 0 1 1-e 0+e 0+e],c2);patch([0 0 1 1-e 0+e 0+e],[0 1 1 1-e 1-e 0+e],c3);plot([0 1 1 0 0],[0 0 1 1 0]);disp('Mux')
  "pd{2,1}" : Outport
      mask Display: e = 0.06;c1 = [120 230 180]/255;c2 = ([120 230 180]+0)/(256+128);c3 = ([120 230 180]+128)/(256+128);patch([0 1 1 0],[0 0 1 1],c1);patch([0 1 1 1-e 1-e 0+e],[0 0 1 1-e 0+e 0+e],c2);patch([0 0 1 1-e 0+e 0+e],[0 1 1 1-e 1-e 0+e],c3);plot([0 1 1 0 0],[0 0 1 1 0]);
  wires:
  mux/1 -> "pd{2,1}"/1
  "p{2}"/1 -> mux/1
